simulink model "Full_System"  (R2026b)
settings: Solver=FixedStepDiscrete  StopTime=0.4  FixedStep=1e-8
values from neighbouring files (symbols this model uses):
  Ts = 1e-8    (= 1e-08)    [params.m]
undefined symbols (not defined in the file or in its folder): filt
libraries: nesl_utility x13, ee_lib x12, fl_lib x11, eePwmGenerator x2, batteryecm_lib x1
settings Model: SimulationMode=accelerator  Creator=KennyBoum-biha  LastModifiedBy=kenny
settings SolverCC: AutoInsertRateTranBlk=on
settings OptimizationCC: DefaultUnderspecifiedDataType=single  DifferentSizesBufferReuse=on  EnhancedBackFolding=on  MaxStackSize=1024  OptimizationCustomize=off  OptimizeBlockOrder=speed
settings DebuggingCC: ParameterTunabilityLossMsg=error
settings HardwareCC: HardwareBoardFeatureSet=SoCBlockset  ProdHWDeviceType=Texas Instruments->C2000  ProdLargestAtomicFloat=None  ProdLargestAtomicInteger=Integer  ProdLongLongMode=on
settings SFSimCC: MATLABDynamicMemAlloc=off
settings RTWCC: DLArmComputeVersion=19.05  Description=Embedded Coder  HardwareBoard=TI Delfino F28379D LaunchPad  SystemTargetFile=ert.tlc  TLCOptions=-aInlineSetEventsForThisBaseRateFcn=TLC_FALSE -aSuppressMultiTaskScheduler=TLC_FALSE -aRateBasedStepFcn=1  TemplateMakefile=ert_default_tmf  Toolchain=Texas Instruments Code Composer Studio (C2000)
settings CodeAppCC: ForceParamTrailComments=on  OperatorAnnotations=on
settings ERTTargetCC: CodeReplacementLibrary=TI C28x  DynamicArrayContainerType=coder::array  ERTCustomFileBanners=off  ExtModeAutomaticAllocSize=off  ExtModeIntrfLevel=Level2 - Open  ExtModeMexFile=ext_xcp  ExtModeStaticAlloc=on  ModelStepFunctionPrototypeControlCompliant=off  SupportContinuousTime=on  SupportNonInlinedSFcns=on
settings SimscapeCC: SimscapeUseEnergyAccounting=off

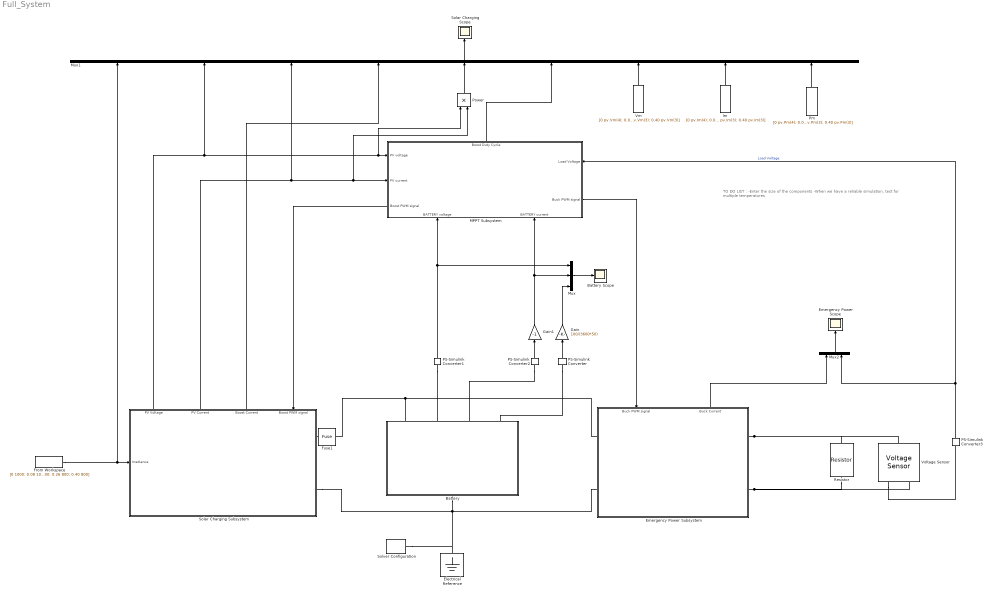
== system Full_System ==
  note: TO DO LIST :
      |
      | -Enter the size of the components
      | -When we have a reliable simulation, test for multiple temperatures
  Battery : Subsystem
      settings: PortSchema="{\"entries\":[{\"content\":{\"sides\":[{\"content\":{},\"type\":\"ConnectorPlacement.EquallySpacedRectSide\",\"uuid\":\"89519b6f-1ccf-4bbb-95e3-dc5788990cfc\"},{\"content\":{\"side\":\"RIGHT\"},\"type\":\"ConnectorPlacement.EquallySpacedRectSide\",\"uuid\":\"d70a0ac1-9e7f-4c7c-9005-64bd181e98b4\"},{\"content\":{\"connectorIds\":[\"LConn1\",\"LConn2\",\"LConn3\",\"LConn4\"],\"side\":\"TOP\"},\"type\":\"ConnectorPlacement.EquallySpacedRectSide\",\"uuid\":\"8f5b6fbc-ab25-4190-a3b5-0819bf7473bb\"},{\"content\":{\"connectorIds\":[\"RConn1\"],\"side\":\"BOTTOM\"},\"type\":\"ConnectorPlacement.EquallySpacedRectSide\",\"uuid\":\"80845846-eb77-420c-a194-e8ea97e2cc30\"}]},\"type\":\"ConnectorPlacement.EquallySpacedConnector\",\"uuid\":\"2b23194f-e17a-4aa0-a4f9-99eaf33779de\"}],\"packageUris\":[\"http://schema.mathworks.com/mf0/Connector/R2020b\"],\"version\":\"1.0\"}"
  Battery Scope : Scope
      settings: ActiveDisplayYMinimum=-6.4437781308415341  ActiveDisplayYMaximum=56.272106347516569  DataLoggingDecimation=50  DataLoggingVariableName=ScopeData2
  Electrical Reference : fl_lib/Electrical/Electrical Elements/Electrical Reference
  Emergency Power Scope : Scope
      settings: ActiveDisplayYMinimum=-0.63228695856137551  ActiveDisplayYMaximum=5.690582635720757  DataLoggingDecimation=50  DataLoggingVariableName=ScopeData2
  Emergency Power Subsystem : Subsystem
      settings: PortSchema="{\"entries\":[{\"content\":{\"sides\":[{\"content\":{\"connectorIds\":[\"LConn1\",\"LConn2\"]},\"type\":\"ConnectorPlacement.EquallySpacedRectSide\",\"uuid\":\"cf3750f3-3e81-4659-820f-f75c62c5389c\"},{\"content\":{\"connectorIds\":[\"RConn1\",\"RConn2\"],\"side\":\"RIGHT\"},\"type\":\"ConnectorPlacement.EquallySpacedRectSide\",\"uuid\":\"3e630a51-3c98-4ea6-b09a-757b6c47ec4c\"},{\"content\":{\"connectorIds\":[\"In1\",\"Out1\"],\"side\":\"TOP\"},\"type\":\"ConnectorPlacement.EquallySpacedRectSide\",\"uuid\":\"d6b0d433-2319-4baf-b8a3-4fb876102fd6\"},{\"content\":{\"side\":\"BOTTOM\"},\"type\":\"ConnectorPlacement.EquallySpacedRectSide\",\"uuid\":\"63ecf188-e0c8-40d8-ac0e-f3629d4410b9\"}]},\"type\":\"ConnectorPlacement.EquallySpacedConnector\",\"uuid\":\"13c5517f-e21d-46a3-ac40-d14bb8a08b57\"}],\"packageUris\":[\"http://schema.mathworks.com/mf0/Connector/R2020b\"],\"version\":\"1.0\"}"
  From Workspace : FromWorkspace  VariableName=[0 1000; 0.08 1000; 0.10 600; 0.16 600; 0.18 400; 0.24 400; 0.26 800; 0.40 800]
  Fuse1 : ee_lib/Switches & Breakers/Fuse  prm=1  I_rated=15 A  melt_margin=1  T_fuse=0 s  I2t=500 A^2*s  I_vec=[1.9, 2, 2.5, 30] A  t_vec=[10000, 1, .3, .001] s  R_closed=0.01 Ohm  G_open=1e-8 1/Ohm  exposemeasurement=ee.enum.exposemeasurement.hidden
  Gain : Gain  Gain=100/(3600*50)
  Gain1 : Gain  Gain=-1
  Im : FromWorkspace  VariableName=[0 pv.Im(4); 0.08 pv.Im(4); 0.10 pv.Im(2); 0.16 pv.Im(2); 0.18 pv.Im(1); 0.24 pv.Im(1); 0.26 pv.Im(3); 0.40 pv.Im(3)]
  MPPT Subsystem : Subsystem
      settings: PortSchema="{\"entries\":[{\"content\":{\"sides\":[{\"content\":{\"connectorIds\":[\"In1\",\"In2\",\"Out3\"]},\"type\":\"ConnectorPlacement.EquallySpacedRectSide\",\"uuid\":\"9861c5ac-f581-4965-b434-078b26985e37\"},{\"content\":{\"connectorIds\":[\"In5\",\"Out1\"],\"side\":\"RIGHT\"},\"type\":\"ConnectorPlacement.EquallySpacedRectSide\",\"uuid\":\"a93de12d-5e32-486a-9221-538754dd8d9c\"},{\"content\":{\"connectorIds\":[\"Out2\"],\"side\":\"TOP\"},\"type\":\"ConnectorPlacement.EquallySpacedRectSide\",\"uuid\":\"228dca20-1858-4fa3-8d58-50b7eb576924\"},{\"content\":{\"connectorIds\":[\"In3\",\"In4\"],\"side\":\"BOTTOM\"},\"type\":\"ConnectorPlacement.EquallySpacedRectSide\",\"uuid\":\"87bfe4fb-7a74-4257-a234-8b691987d317\"}]},\"type\":\"ConnectorPlacement.EquallySpacedConnector\",\"uuid\":\"9c35c19e-5cf1-449e-9944-3961626a0eeb\"}],\"packageUris\":[\"http://schema.mathworks.com/mf0/Connector/R2020b\"],\"version\":\"1.0\"}"
  Mux : Mux  Inputs=3
  Mux1 : Mux  Inputs=9
  Mux2 : Mux  Inputs=2
  PS-Simulink Converter : nesl_utility/PS-Simulink Converter  PhysicalDomain=network_engine_domain  SubClassName=ps_output  LeftPortType=input  RightPortType=output  PseudoPeriodic=off  Frequencies=[]  VectorFormat=inherit  Unit=C  AffineConversion=off
  PS-Simulink Converter1 : nesl_utility/PS-Simulink Converter  PhysicalDomain=network_engine_domain  SubClassName=ps_output  LeftPortType=input  RightPortType=output  PseudoPeriodic=off  Frequencies=[]  VectorFormat=inherit  Unit=V  AffineConversion=off
  PS-Simulink Converter2 : nesl_utility/PS-Simulink Converter  PhysicalDomain=network_engine_domain  SubClassName=ps_output  LeftPortType=input  RightPortType=output  PseudoPeriodic=off  Frequencies=[]  VectorFormat=inherit  Unit=A  AffineConversion=off
  PS-Simulink Converter3 : nesl_utility/PS-Simulink Converter  PhysicalDomain=network_engine_domain  SubClassName=ps_output  LeftPortType=input  RightPortType=output  PseudoPeriodic=off  Frequencies=[]  VectorFormat=inherit  Unit=V  AffineConversion=off
  Pm : FromWorkspace  VariableName=[0 pv.Pm(4); 0.08 pv.Pm(4); 0.10 pv.Pm(2); 0.16 pv.Pm(2); 0.18 pv.Pm(1); 0.24 pv.Pm(1); 0.26 pv.Pm(3); 0.40 pv.Pm(3)]
  Power : Product
  Resistor : fl_lib/Electrical/Electrical Elements/Resistor  R=1.667 Ohm  i_specify=off  i_priority=None  i=0 A  i_nominal_specify=off  i_nominal_value=1  i_nominal_unit=A  v_specify=off  v_priority=None  v=0 V  v_nominal_specify=off  v_nominal_value=1  v_nominal_unit=V
  Solar Charging Scope : Scope
      settings: ActiveDisplayYMinimum=-16.020601094524679  ActiveDisplayYMaximum=115.218057865101  DataLoggingDecimation=50
  Solar Charging Subsystem : Subsystem
      settings: PortSchema="{\"entries\":[{\"content\":{\"sides\":[{\"content\":{\"connectorIds\":[\"In1\"]},\"type\":\"ConnectorPlacement.EquallySpacedRectSide\",\"uuid\":\"cb229151-0742-4502-9ccd-990ff05f6a8c\"},{\"content\":{\"connectorIds\":[\"RConn1\",\"RConn2\"],\"side\":\"RIGHT\"},\"type\":\"ConnectorPlacement.EquallySpacedRectSide\",\"uuid\":\"9e14cc4e-58f0-4588-8f9d-a6a650a5df1b\"},{\"content\":{\"connectorIds\":[\"Out1\",\"Out2\",\"Out3\",\"In2\"],\"side\":\"TOP\"},\"type\":\"ConnectorPlacement.EquallySpacedRectSide\",\"uuid\":\"ec81657c-9ee6-4126-bdd0-5a56d1ba93e0\"},{\"content\":{\"side\":\"BOTTOM\"},\"type\":\"ConnectorPlacement.EquallySpacedRectSide\",\"uuid\":\"af2fcdce-74c3-4fd4-8f62-628e3ce2691d\"}]},\"type\":\"ConnectorPlacement.EquallySpacedConnector\",\"uuid\":\"153089d4-0393-4364-aaa8-7b9cfec9044a\"}],\"packageUris\":[\"http://schema.mathworks.com/mf0/Connector/R2020b\"],\"version\":\"1.0\"}"
  Solver Configuration : nesl_utility/Solver Configuration  PhysicalDomain=network_engine_domain  SubClassName=solver  LeftPortType=input  RightPortType=generic  Tones=[]  Harmonics=[]  SimulateNoise=off  Profile=off  UseLocalSampling=off  EnableSwitchedLinearOptims=on  FrequencyDomain=off  UseCCode=off  RelTol=0.001  AbsTol=0.001  MinStep=1e-09  ToWorkspace=off  RevertToSquareIcSolve=off  NumHomotopyIterations=100  PhasorMode=off  PhasorModeNumHarmonics=1  ConsistencySolver=NEWTON_XTOL_AFTER_FTOL  CanonicalOrdering=CANONICAL  OptimizeIntermediates=OPTIMIZED  MulticoreSolverChoice=BACKWARD_EULER  IndexReductionMethod=DerivativeReplacement  DoDC=off  ResidualTolerance=1e-09  ConsistencyTolSource=GLOBAL  ConsistencyAbsTol=0.001  ConsistencyRelTol=0.001  ConsistencyTolFactor=0.001  UseLocalSolver=on  LocalSolverChoice=NE_BACKWARD_EULER_ADVANCER  ResolveIndetEquations=on  FunctionEvalNumThread=1  LocalSolverSampleTime=Ts  DoFixedCost=on  MaxNonlinIter=3  MaxModeIter=2  ComputeImpulses=off  ImpulseIterations=2  LinearAlgebra=auto  LinearAlgebraNumThread=0  EquationFormulation=NE_TIME_EF  DelaysMemoryBudget=1024  AutomaticFiltering=on  FilteringTimeConstant=0.001  PartitionStorageMethod=AS_NEEDED  PartitionMemoryBudget=1024  PartitionMethod=BALANCED  MultibodyUseLocalSolver=on  MultibodyLocalSolverChoice=ODE1  MultibodyLocalSolverSampleTime=0.001
  Vm : FromWorkspace  VariableName=[0 pv.Vm(4); 0.08 pv.Vm(4); 0.10 pv.Vm(2); 0.16 pv.Vm(2); 0.18 pv.Vm(1); 0.24 pv.Vm(1); 0.26 pv.Vm(3); 0.40 pv.Vm(3)]
  Voltage Sensor : fl_lib/Electrical/Electrical Sensors/Voltage Sensor
  wires:
  Mux/1 -> Battery Scope/1
  Solar Charging Subsystem/1(PV Voltage) -> Mux1/2, MPPT Subsystem/1(PV voltage), Power/1
  Solar Charging Subsystem/2(PV Current) -> Power/2, MPPT Subsystem/2(PV current), Mux1/3
  Mux1/1 -> Solar Charging Scope/1
  PS-Simulink Converter1/1 -> Mux/1, MPPT Subsystem/3(BATTERY voltage)
  PS-Simulink Converter2/1 -> Gain1/1
  Gain/1 -> Mux/3
  Emergency Power Subsystem/1(Buck Current) -> Mux2/1
  Mux2/1 -> Emergency Power Scope/1
  PS-Simulink Converter3/1 -> MPPT Subsystem/5(Load Voltage), Mux2/2  "Load Voltage"
  PS-Simulink Converter/1 -> Gain/1
  MPPT Subsystem/3(Boost PWM signal) -> Solar Charging Subsystem/2(Boost PWM signal)
  MPPT Subsystem/1(Buck PWM signal) -> Emergency Power Subsystem/1(Buck PWM signal)
  MPPT Subsystem/2(Boost Duty Cycle) -> Mux1/6
  Gain1/1 -> Mux/2, MPPT Subsystem/4(BATTERY current)
  From Workspace/1 -> Mux1/1, Solar Charging Subsystem/1(Irradiance)
  Power/1 -> Mux1/5
  Pm/1 -> Mux1/9
  Im/1 -> Mux1/8
  Vm/1 -> Mux1/7
  Solar Charging Subsystem/3(Boost Current) -> Mux1/4
  connections:
  Emergency Power Subsystem/RConn1 -- Voltage Sensor/LConn1 -- Resistor/LConn1
  Emergency Power Subsystem/RConn2 -- Resistor/RConn1 -- Voltage Sensor/RConn2
  Emergency Power Subsystem/LConn2 -- Battery/RConn1 -- Solar Charging Subsystem/RConn2 -- Electrical Reference/LConn1 -- Solver Configuration/RConn1
  Voltage Sensor/RConn1 -- PS-Simulink Converter3/LConn1
  Emergency Power Subsystem/LConn1 -- Battery/LConn1 -- Fuse1/RConn1
  PS-Simulink Converter1/LConn1 -- Battery/LConn2
  PS-Simulink Converter2/LConn1 -- Battery/LConn3
  PS-Simulink Converter/LConn1 -- Battery/LConn4
  Fuse1/LConn1 -- Solar Charging Subsystem/RConn1

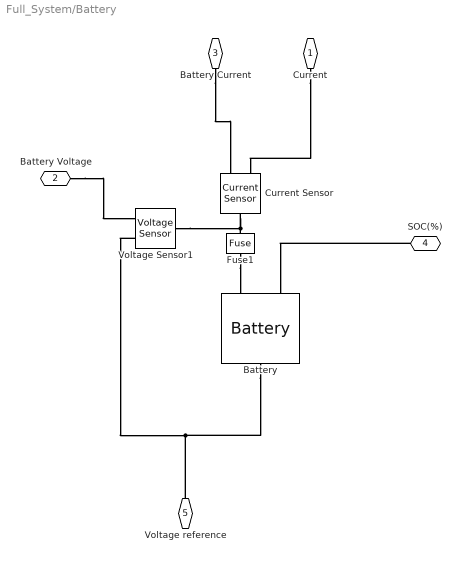
== system Full_System/Battery ==
  Battery : batteryecm_lib/Battery  Vnom=51 V  prm_dir=simscape.enum.battery.prm_dir.disabled  R1_dis=2 Ohm  R1_ch=2 Ohm  R1=0.02 Ohm  prm_AH=simscape.enum.battery.prm_AH.finite  AH=50 A*hr  V1=48.8 V  AH1=20 A*hr  prm_R2=simscape.enum.battery.prm_R2.disabled  R2=2000 Ohm  Tmeas=298.15 K  charge_measurement_port=simscape.enum.battery.enable.yes  prm_dyn=simscape.enum.battery.prm_dyn.off  Rp1=0.005 Ohm  tau1=30 s  Rp2=0.005 Ohm  tau2=30 s  Rp3=0.005 Ohm  tau3=30 s  Rp4=0.005 Ohm  tau4=30 s  Rp5=0.005 Ohm  tau5=30 s  prm_fade=simscape.enum.battery.prm_fade.disabled  N_fade=100  AH_fade=45 A*hr  R1_fade=2.02 Ohm  R1_ch_fade=2.02 Ohm  V1_fade=10.35 V  prm_age=simscape.enum.battery.prm_age.disabled  prm_age_OCV=simscape.enum.battery.prm_age_OCV.OCV  OCV_age=0.9  SOC_age=60  Tmeas_age=298.15 K  delta_time_age_vec=[0] d  temperature_age_vec=[273] K  OCV_scaling_age=2.2134e6  OCV_offset_age=1.632e6  temp_exp_age=0.515833569 V  t_exp_age=0.75  Vnom_T2=12 V  R1_T2=2.2 Ohm  R1_T2_dis=2.2 Ohm  R1_T2_ch=2.2 Ohm  V1_T2=11.4 V  R2_T2=2200 Ohm  Rp1_T2=0.005 Ohm  tau1_T2=30 s  Rp2_T2=0.005 Ohm  tau2_T2=30 s  Rp3_T2=0.005 Ohm  tau3_T2=30 s  Rp4_T2=0.005 Ohm  tau4_T2=30 s  Rp5_T2=0.005 Ohm  tau5_T2=30 s  Tmeas2=273.15 K  thermal_port=simscape.enum.thermaleffects.omit  thermal_mass=30000 J/K  i_specify=off  i_priority=None  i=0 A  i_nominal_specify=off  i_nominal_value=1  i_nominal_unit=A  v_specify=off  v_priority=None  v=0 V  v_nominal_specify=on  v_nominal_value=1  v_nominal_unit=V  charge_specify=on  charge_priority=High  charge=25 A*hr  charge_nominal_specify=on  charge_nominal_value=1  charge_nominal_unit=A*hr  num_cycles_specify=off  num_cycles_priority=High  num_cycles=0  num_cycles_nominal_specify=off  num_cycles_nominal_value=1  num_cycles_nominal_unit=1  temperature_specify=off  temperature_priority=High  temperature=298.15 K  temperature_nominal_specify=off  temperature_nominal_value=1  temperature_nominal_unit=K
  Current Sensor : fl_lib/Electrical/Electrical Sensors/Current Sensor
  Fuse1 : ee_lib/Switches & Breakers/Fuse  prm=1  I_rated=60 A  melt_margin=1  T_fuse=0 s  I2t=20000 A^2*s  I_vec=[1.9, 2, 2.5, 30] A  t_vec=[10000, 1, .3, .001] s  R_closed=0.01 Ohm  G_open=1e-8 1/Ohm  exposemeasurement=ee.enum.exposemeasurement.hidden
  Voltage Sensor1 : fl_lib/Electrical/Electrical Sensors/Voltage Sensor
  Current : PMIOPort  Side=Left
  Battery Voltage : PMIOPort  Port=2  Side=Left
  Battery Current : PMIOPort  Port=3  Side=Left
  SOC(%) : PMIOPort  Port=4  Side=Left
  Voltage reference : PMIOPort  Port=5  Side=Right
  connections:
  Voltage Sensor1/LConn1 -- Fuse1/LConn1 -- Current Sensor/LConn1
  SOC(%)/RConn1 -- Battery/LConn2
  Current/RConn1 -- Current Sensor/RConn2
  Battery Current/RConn1 -- Current Sensor/RConn1
  Fuse1/RConn1 -- Battery/LConn1
  Battery Voltage/RConn1 -- Voltage Sensor1/RConn1
  Voltage reference/RConn1 -- Voltage Sensor1/RConn2 -- Battery/RConn1

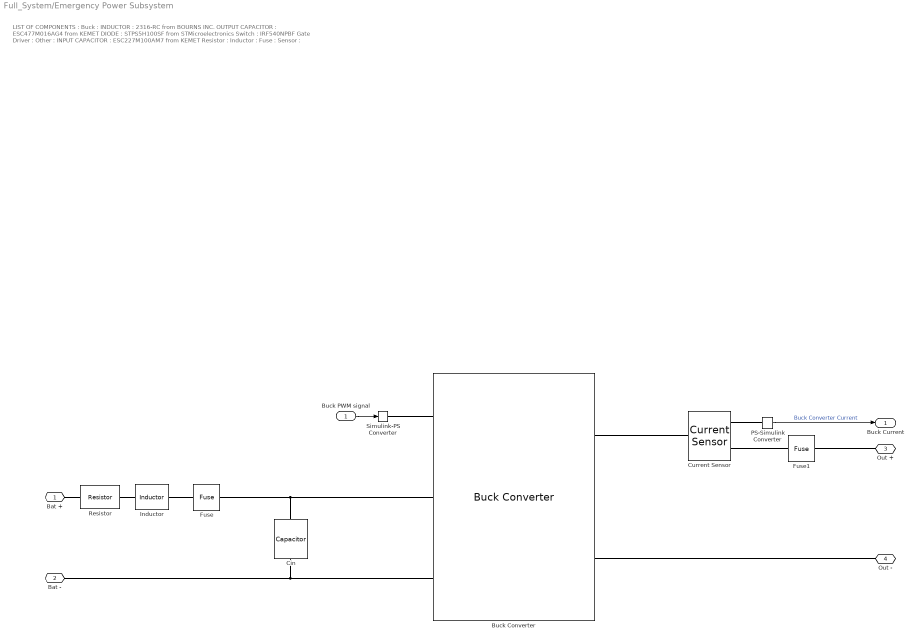
== system Full_System/Emergency Power Subsystem ==
  note: LIST OF COMPONENTS :
      |
      | Buck :
      |
      | INDUCTOR : 2316-RC from BOURNS INC.
      |
      | OUTPUT CAPACITOR : ESC477M016AG4 from KEMET
      |
      | DIODE : STPS5H100SF from STMicroelectronics
      |
      | Switch : IRF540NPBF
      |
      | Gate Driver :
      |
      | Other :
      |
      | INPUT CAPACITOR : ESC227M100AM7 from KEMET
      |
      | Resistor :
      |
      | Inductor :
      |
      | Fuse :
      |
      | Sensor :
  Buck PWM signal : Inport
  Buck Converter : ee_lib/Semiconductors & Converters/Converters/Buck Converter  port_option=ee.enum.controlport.ps  device_type=ee.enum.converters.switchingdevice.ideal  Vf=0.8 V  Ron=0.001 Ohm  Rds=0.001 Ohm  Goff=1e-5 1/Ohm  Vgt=1 V  Vgt_off=-1 V  Ih=1 A  Vth=0.5 V  K=0  diode_param=ee.enum.converters.protectiondiode.nodynamics  diode_Vf=0.7 V  diode_Ron=0.020 Ohm  diode_Goff=3.5e-8 1/Ohm  diode_C=50 nF  diode_iRM=-235 A  diode_iF=300 A  diode_idot=-50 A/us  diode_trr_param=ee.enum.converters.diodetrr.trr_factor  diode_trr_factor=3  diode_trr=15 us  diode_Qrr=1500 s*uA  Lf=220e-6 H  Rl=0.054 Ohm  Cf=470e-6 F  Rf=0.2 Ohm  snubber_type=ee.enum.converters.snubber.exclude  Cs=1e-7 F  Rs=0.1 Ohm  iL_specify=on  iL_priority=High  iL=0 A  iL_nominal_specify=off  iL_nominal_value=1  iL_nominal_unit=A  vc_specify=on  vc_priority=High  vc=0 V  vc_nominal_specify=off  vc_nominal_value=1  vc_nominal_unit=V
  Cin : ee_lib/Passive/Capacitor  cap_option=ee.enum.passive.capacitor.capOption.const  c=220e-6 F  Cvec=[1e-05, 1e-06] F  Vvec=[0, 10] V  CV_table_symmetry=ee.enum.passive.capacitor.tableSymmetry.yes  f_vec=[1, 10] kHz  DFext_vec=[.8, 1.2]  enable_C_tol=ee.enum.toleranceApplication.none  averaging_period=0 s  C_tol=5  tol_distribution=ee.enum.toleranceDistribution.uniform  nSigma=4  r=0.2 Ohm  g=0 1/Ohm  enable_operating_limits=ee.enum.enable.no  operating_limit_action=ee.enum.passive.reportOpLim.warn  max_working_voltage_range=[-25, 25] V  power_rating=1 W  maxTemperature=85 degC  thermalEnable=false  thermalMass=1 J/K  i_specify=off  i_priority=None  i=0 A  i_nominal_specify=off  i_nominal_value=1  i_nominal_unit=A  v_specify=off  v_priority=None  v=0 V  v_nominal_specify=off  v_nominal_value=1  v_nominal_unit=V  vc_specify=on  vc_priority=High  vc=49.5 V  vc_nominal_specify=off  vc_nominal_value=1  vc_nominal_unit=V  T_specify=off  T_priority=None  T=298.15 K  T_nominal_specify=off  T_nominal_value=1  T_nominal_unit=K
  Current Sensor : fl_lib/Electrical/Electrical Sensors/Current Sensor
  Fuse : ee_lib/Switches & Breakers/Fuse  prm=1  I_rated=15 A  melt_margin=1  T_fuse=0 s  I2t=500 A^2*s  I_vec=[1.9, 2, 2.5, 30] A  t_vec=[10000, 1, .3, .001] s  R_closed=0.01 Ohm  G_open=1e-8 1/Ohm  exposemeasurement=ee.enum.exposemeasurement.hidden
  Fuse1 : ee_lib/Switches & Breakers/Fuse  prm=1  I_rated=25 A  melt_margin=1  T_fuse=0 s  I2t=2000 A^2*s  I_vec=[1.9, 2, 2.5, 30] A  t_vec=[10000, 1, .3, .001] s  R_closed=0.01 Ohm  G_open=1e-8 1/Ohm  exposemeasurement=ee.enum.exposemeasurement.hidden
  Inductor : ee_lib/Passive/Inductor  l=1e-6 H  enable_L_tol=ee.enum.toleranceApplication.none  L_tol=20  tol_distribution=ee.enum.toleranceDistribution.uniform  nSigma=4  r=0 Ohm  g=1e-9 1/Ohm  enable_operating_limits=ee.enum.enable.no  operating_limit_action=ee.enum.passive.reportOpLim.warn  max_working_current=1 A  power_rating=1 W  i_L_specify=off  i_L_priority=High  i_L=0 A  i_L_nominal_specify=off  i_L_nominal_value=1  i_L_nominal_unit=A
  PS-Simulink Converter : nesl_utility/PS-Simulink Converter  PhysicalDomain=network_engine_domain  SubClassName=ps_output  LeftPortType=input  RightPortType=output  PseudoPeriodic=off  Frequencies=[]  VectorFormat=inherit  Unit=A  AffineConversion=off
  Resistor : fl_lib/Electrical/Electrical Elements/Resistor  R=0.02 Ohm  i_specify=off  i_priority=None  i=0 A  i_nominal_specify=off  i_nominal_value=1  i_nominal_unit=A  v_specify=off  v_priority=None  v=0 V  v_nominal_specify=off  v_nominal_value=1  v_nominal_unit=V
  Simulink-PS Converter : nesl_utility/Simulink-PS Converter  PhysicalDomain=network_engine_domain  SubClassName=ps_input  LeftPortType=input  RightPortType=output  PseudoPeriodic=off  Frequencies=[]  NoiseDistribution=none  NoiseParameters=[]  Unit=V  AffineConversion=off  FilteringAndDerivatives=provide  SimscapeFilterOrder=1  InputFilterTimeConstant=0.001  UdotUserProvided=0
  Bat + : PMIOPort  Side=Left
  Bat - : PMIOPort  Port=2  Side=Left
  Out + : PMIOPort  Port=3  Side=Right
  Out - : PMIOPort  Port=4  Side=Right
  Buck Current : Outport
  wires:
  PS-Simulink Converter/1 -> Buck Current/1  "Buck Converter Current"
  Buck PWM signal/1 -> Simulink-PS Converter/1
  connections:
  Buck Converter/LConn2 -- Fuse/RConn1 -- Cin/LConn1
  Current Sensor/LConn1 -- Buck Converter/RConn1
  Bat -/RConn1 -- Buck Converter/LConn3 -- Cin/RConn1
  Out -/RConn1 -- Buck Converter/RConn2
  PS-Simulink Converter/LConn1 -- Current Sensor/RConn1
  Fuse/LConn1 -- Inductor/RConn1
  Fuse1/LConn1 -- Current Sensor/RConn2
  Fuse1/RConn1 -- Out +/RConn1
  Simulink-PS Converter/RConn1 -- Buck Converter/LConn1
  Resistor/LConn1 -- Bat +/RConn1
  Inductor/LConn1 -- Resistor/RConn1

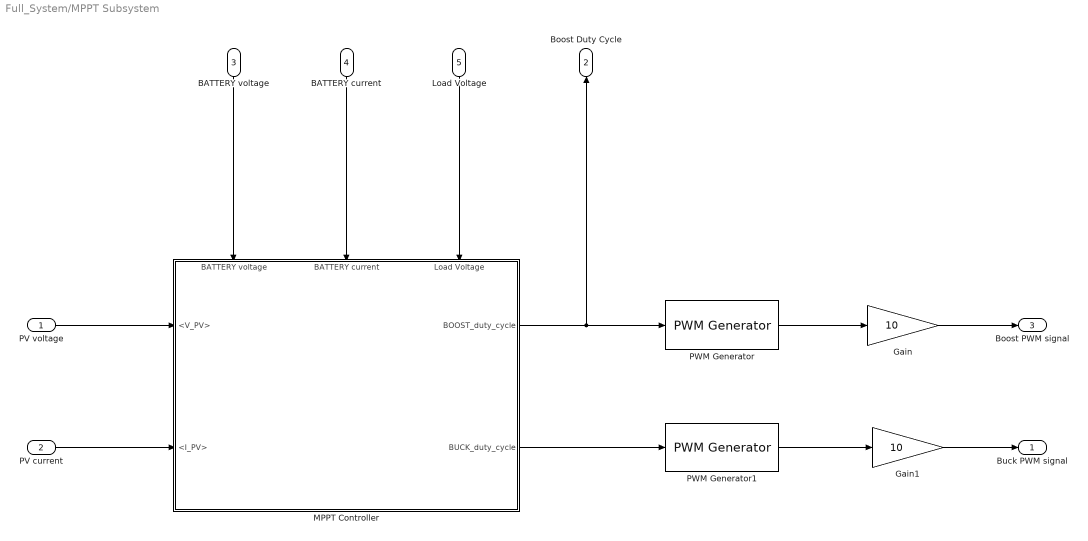
== system Full_System/MPPT Subsystem ==
  PV voltage : Inport
  PV current : Inport  Port=2
  BATTERY voltage : Inport  Port=3
  BATTERY current : Inport  Port=4
  Load Voltage : Inport  Port=5
  Gain : Gain  Gain=10
  Gain1 : Gain  Gain=10
  MPPT Controller : Subsystem
      settings: PortSchema="{\"entries\":[{\"content\":{\"sides\":[{\"content\":{\"connectorIds\":[\"In1\",\"In2\"]},\"type\":\"ConnectorPlacement.EquallySpacedRectSide\",\"uuid\":\"28e1e1ab-227c-4724-b0c4-35db6fee0cc0\"},{\"content\":{\"connectorIds\":[\"Out1\",\"Out2\"],\"side\":\"RIGHT\"},\"type\":\"ConnectorPlacement.EquallySpacedRectSide\",\"uuid\":\"63eff4b4-ca4f-48d2-8ac3-b8c12c25396e\"},{\"content\":{\"connectorIds\":[\"In3\",\"In4\",\"In5\"],\"side\":\"TOP\"},\"type\":\"ConnectorPlacement.EquallySpacedRectSide\",\"uuid\":\"2071d001-f4a1-4b01-bdc1-637c633b064a\"}]},\"type\":\"ConnectorPlacement.EquallySpacedConnector\",\"uuid\":\"cda405f3-33c0-4e2c-948a-359ae1570125\"}],\"packageUris\":[\"http://schema.mathworks.com/mf0/Connector/R2020b\"],\"version\":\"1.0\"}"
  PWM Generator : eePwmGenerator/PWM Generator  CarrCount=Up  Tper=20e-6  Tdelay=0  Ts=Ts
  PWM Generator1 : eePwmGenerator/PWM Generator  CarrCount=Up  Tper=20e-6  Tdelay=0  Ts=Ts
  Buck PWM signal : Outport
  Boost Duty Cycle : Outport  Port=2
  Boost PWM signal : Outport  Port=3
  wires:
  PWM Generator/1 -> Gain/1
  PV voltage/1 -> MPPT Controller/1(<V_PV>)
  MPPT Controller/1(BOOST_duty_cycle) -> Boost Duty Cycle/1, PWM Generator/1
  PV current/1 -> MPPT Controller/2(<I_PV>)
  BATTERY voltage/1 -> MPPT Controller/3(BATTERY voltage)
  BATTERY current/1 -> MPPT Controller/4(BATTERY current)
  MPPT Controller/2(BUCK_duty_cycle) -> PWM Generator1/1
  Gain1/1 -> Buck PWM signal/1
  PWM Generator1/1 -> Gain1/1
  Load Voltage/1 -> MPPT Controller/5(Load Voltage)
  Gain/1 -> Boost PWM signal/1

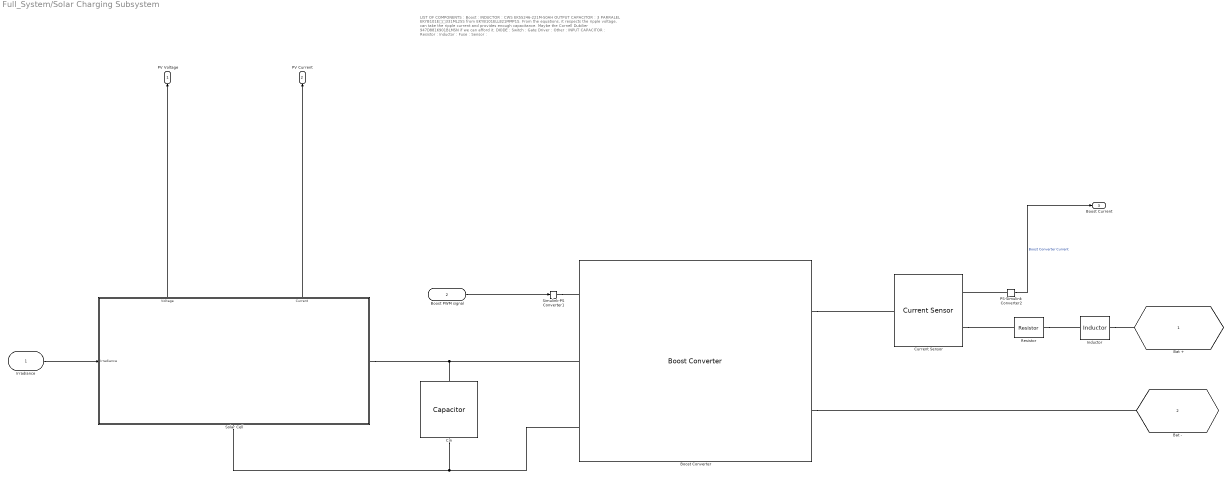
== system Full_System/Solar Charging Subsystem ==
  note: LIST OF COMPONENTS :
      |
      | Boost :
      |
      | INDUCTOR : CWS EK55246-221M-50AH
      |
      | OUTPUT CAPACITOR : 3 PARRALEL EKYB101E□□331ML25S from EKYB101ELL821MMP1S. From the equations, it respects the ripple voltage, can take the ripple current and provides enough capacitance. Maybe the Cornell Dubilier 947D881K901BLMSN if we can afford it.
      |
      | DIODE :
      |
      | Switch :
      |
      | Gate Driver :
      |
      | Other :
      |
      | INPUT CAPACITOR :
      |
      | Resistor :
      |
      | Inductor :
      |
      | Fuse :
      |
      | Sensor :
  Irradiance : Inport
  Boost PWM signal : Inport  Port=2
  Boost Converter : ee_lib/Semiconductors & Converters/Converters/Boost Converter  port_option=ee.enum.controlport.ps  device_type=ee.enum.converters.switchingdevice.ideal  Vf=0.8 V  Ron=0.001 Ohm  Rds=0.001 Ohm  Goff=1e-5 1/Ohm  Vgt=1 V  Vgt_off=-1 V  Ih=1 A  Vth=0.5 V  K=0  diode_param=ee.enum.converters.protectiondiode.nodynamics  diode_Vf=0.8 V  diode_Ron=0.001 Ohm  diode_Goff=1e-5 1/Ohm  diode_C=50 nF  diode_iRM=-235 A  diode_iF=300 A  diode_idot=-50 A/us  diode_trr_param=ee.enum.converters.diodetrr.trr_factor  diode_trr_factor=3  diode_trr=15 us  diode_Qrr=1500 s*uA  Lf=220e-6 H  Rl=0 Ohm  Cf=990e-6 F  Rf=0.0093 Ohm  snubber_type=ee.enum.converters.snubber.exclude  Cs=1e-7 F  Rs=0.1 Ohm  iL_specify=on  iL_priority=High  iL=0 A  iL_nominal_specify=off  iL_nominal_value=1  iL_nominal_unit=A  vc_specify=on  vc_priority=High  vc=49.5 V  vc_nominal_specify=off  vc_nominal_value=1  vc_nominal_unit=V
  Cin : ee_lib/Passive/Capacitor  cap_option=ee.enum.passive.capacitor.capOption.const  c=220e-6 F  Cvec=[1e-05, 1e-06] F  Vvec=[0, 10] V  CV_table_symmetry=ee.enum.passive.capacitor.tableSymmetry.yes  f_vec=[1, 10] kHz  DFext_vec=[.8, 1.2]  enable_C_tol=ee.enum.toleranceApplication.none  averaging_period=0 s  C_tol=5  tol_distribution=ee.enum.toleranceDistribution.uniform  nSigma=4  r=0.2 Ohm  g=0 1/Ohm  enable_operating_limits=ee.enum.enable.no  operating_limit_action=ee.enum.passive.reportOpLim.warn  max_working_voltage_range=[-25, 25] V  power_rating=1 W  maxTemperature=85 degC  thermalEnable=false  thermalMass=1 J/K  i_specify=off  i_priority=None  i=0 A  i_nominal_specify=off  i_nominal_value=1  i_nominal_unit=A  v_specify=off  v_priority=None  v=0 V  v_nominal_specify=off  v_nominal_value=1  v_nominal_unit=V  vc_specify=on  vc_priority=High  vc=27 V  vc_nominal_specify=off  vc_nominal_value=1  vc_nominal_unit=V  T_specify=off  T_priority=None  T=298.15 K  T_nominal_specify=off  T_nominal_value=1  T_nominal_unit=K
  Current Sensor : fl_lib/Electrical/Electrical Sensors/Current Sensor
  Inductor : ee_lib/Passive/Inductor  l=1e-6 H  enable_L_tol=ee.enum.toleranceApplication.none  L_tol=20  tol_distribution=ee.enum.toleranceDistribution.uniform  nSigma=4  r=0 Ohm  g=1e-9 1/Ohm  enable_operating_limits=ee.enum.enable.no  operating_limit_action=ee.enum.passive.reportOpLim.warn  max_working_current=1 A  power_rating=1 W  i_L_specify=off  i_L_priority=High  i_L=0 A  i_L_nominal_specify=off  i_L_nominal_value=1  i_L_nominal_unit=A
  PS-Simulink Converter2 : nesl_utility/PS-Simulink Converter  PhysicalDomain=network_engine_domain  SubClassName=ps_output  LeftPortType=input  RightPortType=output  PseudoPeriodic=off  Frequencies=[]  VectorFormat=inherit  Unit=A  AffineConversion=off
  Resistor : fl_lib/Electrical/Electrical Elements/Resistor  R=0.02 Ohm  i_specify=off  i_priority=None  i=0 A  i_nominal_specify=off  i_nominal_value=1  i_nominal_unit=A  v_specify=off  v_priority=None  v=0 V  v_nominal_specify=off  v_nominal_value=1  v_nominal_unit=V
  Simulink-PS Converter1 : nesl_utility/Simulink-PS Converter  PhysicalDomain=network_engine_domain  SubClassName=ps_input  LeftPortType=input  RightPortType=output  PseudoPeriodic=off  Frequencies=[]  NoiseDistribution=none  NoiseParameters=[]  Unit=V  AffineConversion=off  FilteringAndDerivatives=provide  SimscapeFilterOrder=1  InputFilterTimeConstant=0.001  UdotUserProvided=0
  Solar Cell : Subsystem
      settings: PortSchema="{\"entries\":[{\"content\":{\"sides\":[{\"content\":{\"connectorIds\":[\"In1\"]},\"type\":\"ConnectorPlacement.EquallySpacedRectSide\",\"uuid\":\"a365bae5-cf10-4a4f-8e40-ff085d2edea1\"},{\"content\":{\"connectorIds\":[\"RConn1\"],\"side\":\"RIGHT\"},\"type\":\"ConnectorPlacement.EquallySpacedRectSide\",\"uuid\":\"97e221b8-f9cd-4f5f-aeff-ebeac244023a\"},{\"content\":{\"connectorIds\":[\"Out1\",\"Out2\"],\"side\":\"TOP\"},\"type\":\"ConnectorPlacement.EquallySpacedRectSide\",\"uuid\":\"67a250c4-1569-4196-ad22-f6520136c2ad\"},{\"content\":{\"connectorIds\":[\"RConn2\"],\"side\":\"BOTTOM\"},\"type\":\"ConnectorPlacement.EquallySpacedRectSide\",\"uuid\":\"153e65b8-deac-4f4c-ad00-32101b9f7a4c\"}]},\"type\":\"ConnectorPlacement.EquallySpacedConnector\",\"uuid\":\"23ef3248-3080-4e87-b3af-c5b83fa8f60a\"}],\"packageUris\":[\"http://schema.mathworks.com/mf0/Connector/R2020b\"],\"version\":\"1.0\"}"
  Bat + : PMIOPort  Side=Right
  Bat - : PMIOPort  Port=2  Side=Right
  PV Voltage : Outport
  PV Current : Outport  Port=2
  Boost Current : Outport  Port=3
  wires:
  PS-Simulink Converter2/1 -> Boost Current/1  "Boost Converter Current"
  Irradiance/1 -> Solar Cell/1(Irradiance)
  Solar Cell/1(Voltage) -> PV Voltage/1
  Solar Cell/2(Current) -> PV Current/1
  Boost PWM signal/1 -> Simulink-PS Converter1/1
  connections:
  Current Sensor/RConn2 -- Resistor/LConn1
  Boost Converter/RConn1 -- Current Sensor/LConn1
  Boost Converter/RConn2 -- Bat -/RConn1
  Cin/RConn1 -- Solar Cell/RConn2 -- Boost Converter/LConn3
  PS-Simulink Converter2/LConn1 -- Current Sensor/RConn1
  Boost Converter/LConn2 -- Solar Cell/RConn1 -- Cin/LConn1
  Simulink-PS Converter1/RConn1 -- Boost Converter/LConn1
  Inductor/RConn1 -- Bat +/RConn1
  Resistor/RConn1 -- Inductor/LConn1

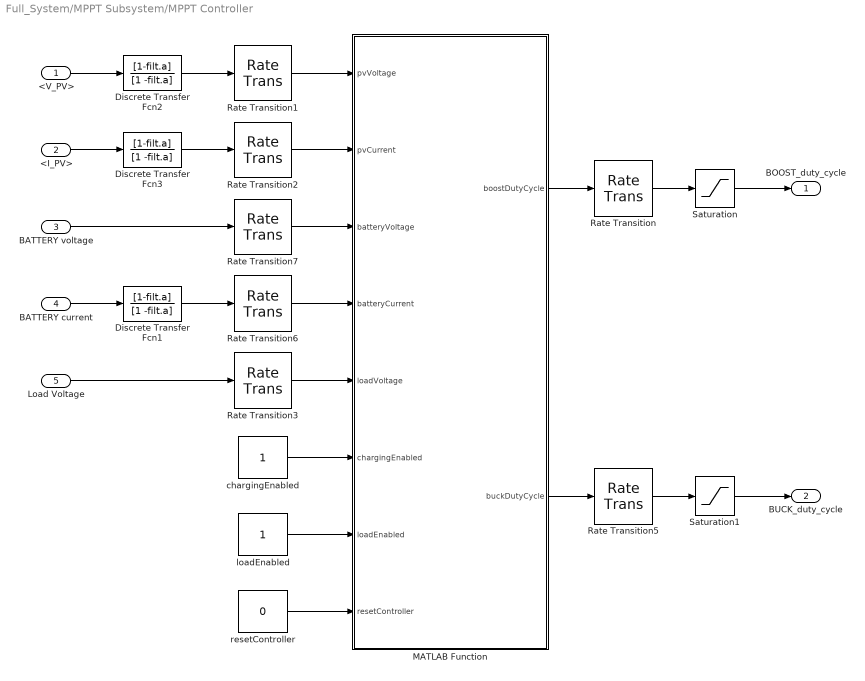
== system Full_System/MPPT Subsystem/MPPT Controller ==
  <V_PV> : Inport
  <I_PV> : Inport  Port=2
  BATTERY voltage : Inport  Port=3
  BATTERY current : Inport  Port=4
  Load Voltage : Inport  Port=5
  Discrete Transfer Fcn1 : DiscreteTransferFcn  Numerator=[1-filt.a]  Denominator=[1 -filt.a]
  Discrete Transfer Fcn2 : DiscreteTransferFcn  Numerator=[1-filt.a]  Denominator=[1 -filt.a]
  Discrete Transfer Fcn3 : DiscreteTransferFcn  Numerator=[1-filt.a]  Denominator=[1 -filt.a]
  MATLAB Function : MATLAB Function  InitFcn=params  TreatAsAtomicUnit=on
  Rate Transition : RateTransition  OutPortSampleTime=Ts
  Rate Transition{1..3,6..7} (5 alike) : RateTransition  OutPortSampleTime=10e-6
  Rate Transition5 : RateTransition  OutPortSampleTime=Ts
  Saturation : Saturate  UpperLimit=0.95  LowerLimit=0
  Saturation1 : Saturate  UpperLimit=0.95  LowerLimit=0
  chargingEnabled : Constant
  loadEnabled : Constant
  resetController : Constant  Value=0
  BOOST_duty_cycle : Outport
  BUCK_duty_cycle : Outport  Port=2
  wires:
  MATLAB Function/1(boostDutyCycle) -> Rate Transition/1
  Discrete Transfer Fcn3/1 -> Rate Transition2/1
  Discrete Transfer Fcn2/1 -> Rate Transition1/1
  <V_PV>/1 -> Discrete Transfer Fcn2/1
  <I_PV>/1 -> Discrete Transfer Fcn3/1
  Saturation/1 -> BOOST_duty_cycle/1
  Rate Transition2/1 -> MATLAB Function/2(pvCurrent)
  Rate Transition1/1 -> MATLAB Function/1(pvVoltage)
  BATTERY voltage/1 -> Rate Transition7/1
  BATTERY current/1 -> Discrete Transfer Fcn1/1
  chargingEnabled/1 -> MATLAB Function/6(chargingEnabled)
  loadEnabled/1 -> MATLAB Function/7(loadEnabled)
  resetController/1 -> MATLAB Function/8(resetController)
  MATLAB Function/2(buckDutyCycle) -> Rate Transition5/1
  Discrete Transfer Fcn1/1 -> Rate Transition6/1
  Rate Transition6/1 -> MATLAB Function/4(batteryCurrent)
  Rate Transition7/1 -> MATLAB Function/3(batteryVoltage)
  Rate Transition3/1 -> MATLAB Function/5(loadVoltage)
  Load Voltage/1 -> Rate Transition3/1
  Rate Transition/1 -> Saturation/1
  Rate Transition5/1 -> Saturation1/1
  Saturation1/1 -> BUCK_duty_cycle/1

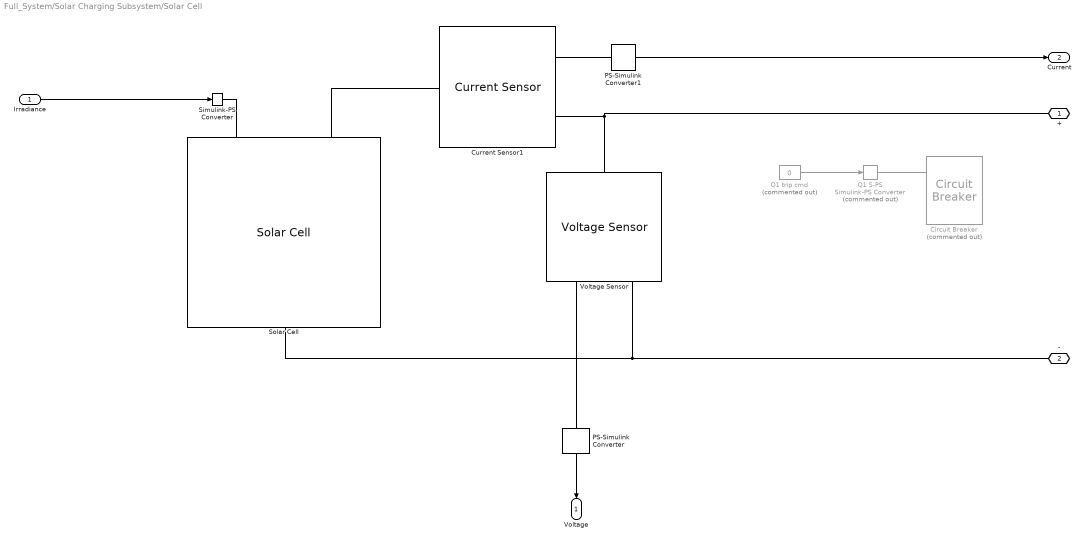
== system Full_System/Solar Charging Subsystem/Solar Cell ==
  Irradiance : Inport
  Circuit Breaker : ee_lib/Switches & Breakers/Circuit Breaker  Commented=on  R_closed=0.001 Ohm  G_open=1e-6 1/Ohm  threshold=0.5 V  breaker_behavior=ee.enum.switches.breakerBehavior.zeroCrossingEnable  port_option=ee.enum.threePhasePort.composite  control_port_option=ee.enum.controlport.ps  i_th=1e-8 A
  Current Sensor1 : fl_lib/Electrical/Electrical Sensors/Current Sensor
  PS-Simulink Converter : nesl_utility/PS-Simulink Converter  PhysicalDomain=network_engine_domain  SubClassName=ps_output  LeftPortType=input  RightPortType=output  PseudoPeriodic=off  Frequencies=[]  VectorFormat=inherit  Unit=V  AffineConversion=off
  PS-Simulink Converter1 : nesl_utility/PS-Simulink Converter  PhysicalDomain=network_engine_domain  SubClassName=ps_output  LeftPortType=input  RightPortType=output  PseudoPeriodic=off  Frequencies=[]  VectorFormat=inherit  Unit=A  AffineConversion=off
  Q1 S-PS : nesl_utility/Simulink-PS Converter  Commented=on  PhysicalDomain=network_engine_domain  SubClassName=ps_input  LeftPortType=input  RightPortType=output  PseudoPeriodic=off  Frequencies=[]  NoiseDistribution=none  NoiseParameters=[]  Unit=1  AffineConversion=off  FilteringAndDerivatives=provide  SimscapeFilterOrder=1  InputFilterTimeConstant=0.001  UdotUserProvided=0
  Q1 trip cmd : Constant  Commented=on  Value=0
  Simulink-PS Converter : nesl_utility/Simulink-PS Converter  PhysicalDomain=network_engine_domain  SubClassName=ps_input  LeftPortType=input  RightPortType=output  PseudoPeriodic=off  Frequencies=[]  NoiseDistribution=none  NoiseParameters=[]  Unit=W/m^2  AffineConversion=off  FilteringAndDerivatives=provide  SimscapeFilterOrder=1  InputFilterTimeConstant=0.001  UdotUserProvided=0
  Solar Cell : ee_lib/Sources/Solar Cell  prm=ee.enum.sources.solar_cell_prm.datasheet  Isc=4.375 A  Voc=0.700 V  Is=1e-6 A  Is2=0 A  Iph=7.34 A  Ir0=1000 W/m^2  ec=1.12615  N2=2  Rs=0.00274428 Ohm  Rp=inf Ohm  N_series=40  N_parallel=2  TIPH1=0.00048 1/K  EG=1.11 eV  TXIS1=3  TXIS2=3  TRS1=0  TRP1=0  Tmeas=25 degC  TFIXED=25 degC  thermal_mass=100 J/K  initial_temperature=25 degC
  Voltage Sensor : fl_lib/Electrical/Electrical Sensors/Voltage Sensor
  + : PMIOPort  Side=Right
  - : PMIOPort  Port=2  Side=Right
  Voltage : Outport
  Current : Outport  Port=2
  wires:
  PS-Simulink Converter1/1 -> Current/1
  Q1 trip cmd/1 -> Q1 S-PS/1
  Irradiance/1 -> Simulink-PS Converter/1
  PS-Simulink Converter/1 -> Voltage/1
  connections:
  Solar Cell/LConn2 -- Current Sensor1/LConn1
  Current Sensor1/RConn1 -- PS-Simulink Converter1/LConn1
  Solar Cell/LConn1 -- Simulink-PS Converter/RConn1
  Q1 S-PS/RConn1 -- Circuit Breaker/LConn1
  PS-Simulink Converter/LConn1 -- Voltage Sensor/RConn1
  Voltage Sensor/RConn2 -- -/RConn1 -- Solar Cell/RConn1
  Voltage Sensor/LConn1 -- Current Sensor1/RConn2 -- +/RConn1

== matlab function Full_System/MPPT Subsystem/MPPT Controller/MATLAB Function ==
  data: pvVoltage input; boostDutyCycle output; pvCurrent input; batteryVoltage input; batteryCurrent input; loadVoltage input; chargingEnabled input; loadEnabled input; resetController input; buckDutyCycle output
function [boostDutyCycle, buckDutyCycle] = MPPT_Algorithm(pvVoltage, pvCurrent, batteryVoltage, batteryCurrent, loadVoltage, chargingEnabled, loadEnabled, resetController)
[boostDutyCycle, buckDutyCycle] = solar_charge_controller(pvVoltage, pvCurrent, batteryVoltage, batteryCurrent, loadVoltage, chargingEnabled, loadEnabled, resetController);

% function DutyCycle = fcn(V, I, mppt)
% DutyCycle = mppt_po(V, I, mppt.Du, mppt.D0, mppt.Dmin, mppt.Dmax);
